simulink model "Spring_Test"  (R2025a)
settings: Solver=ode23t  StartTime=0.0  StopTime=15  RelTol=1e-3  EnableMultiTasking=on
InitFcn:
  | warning off Simulink:SL_MatchingFromNotFound
  | m=1;
  | b=1;
  | k=1;
libraries: fl_lib x15, nesl_utility x4, Custom_lib x1
Description:
  | Copyright 2015-2025 The MathWorks, Inc.
settings Model: Creator=tegel  LastModifiedBy=smiller
settings SolverCC: AlgebraicLoopSolver=TrustRegion
settings DataIOCC: LimitDataPoints=on  SaveFormat=Array  SignalLoggingSaveFormat=ModelDataLogs  ReturnWorkspaceOutputs=off
settings OptimizationCC: ReuseModelBlockBuffer=off  ExpressionDepthLimit=2147483647.0  InitFltsAndDblsToZero=on  LifeSpan=inf
settings DebuggingCC: SaveWithParameterizedLinksMsg=none  UnderspecifiedInitializationDetection=Classic  MergeDetectMultiDrivingBlocksExec=none  FcnCallInpInsideContextMsg=warning  UnconnectedInputMsg=warning  UnconnectedOutputMsg=warning  UnconnectedLineMsg=warning  AllowSymbolicDim=off  StateNameClashWarn=warning  PregeneratedLibrarySubsystemCodeDiagnostic=none  SFUnexpectedBacktrackingDiag=warning  SFNoUnconditionalDefaultTransitionDiag=warning  SFExecutionAtInitializationDiag=none  ArithmeticOperatorsInVariantConditions=warning
settings HardwareCC: ProdBitPerPointer=32.0  ProdBitPerSizeT=32.0  ProdBitPerPtrDiffT=32.0  ProdLargestAtomicFloat=None  ProdIntDivRoundTo=Undefined  ProdEndianess=Unspecified  ProdWordSize=32.0  ProdHWDeviceType=32-bit Generic
settings ModelReferenceCC: EnableRefExpFcnMdlSchedulingChecks=on  PropagateSignalLabelsOutOfModel=off
settings SFSimCC: SimUseLocalCustomCode=off  CustomCodeUndefinedFunction=UseInterfaceOnly
settings RTWCC: RTWUseLocalCustomCode=off  GPUComputeCapability=3.5  DLArmComputeVersion=19.05
settings CodeAppCC: StateflowObjectComments=on
settings GRTTargetCC: TargetFcnLib=ansi_tfl_tmw.mat  TargetLangStandard=C89/C90 (ANSI)  CombineOutputUpdateFcns=off  GRTInterface=on
settings ConfigComp: CovMetricSettings=dw  CovSaveCumulativeToWorkspaceVar=on  CovSaveSingleToWorkspaceVar=on  CovExternalEMLEnable=off  CovSFcnEnable=off
settings SimscapeCC: SimscapeNormalizeSystem=off  SimscapeNominalValues="[{\"value\":\"10\",\"unit\":\"V\"},{\"value\":\"1\",\"unit\":\"A\"},{\"value\":\"10\",\"unit\":\"N*m\"},{\"value\":\"10\",\"unit\":\"bar\"},{\"value\":\"100\",\"unit\":\"kJ/kg\"},{\"value\":\"1\",\"unit\":\"kW\"},{\"value\":\"300\",\"unit\":\"K\"},{\"value\":\"100\",\"unit\":\"cm^3/s\"},{\"value\":\"1\",\"unit\":\"kN\"},{\"value\":\"1\",\"unit\":\"g/cm^3\"},{\"value\":\"1\",\"unit\":\"l\"},{\"value\":\"1\",\"unit\":\"cm^2\"},{\"value\":\"60\",\"unit\":\"Hz\"}]"

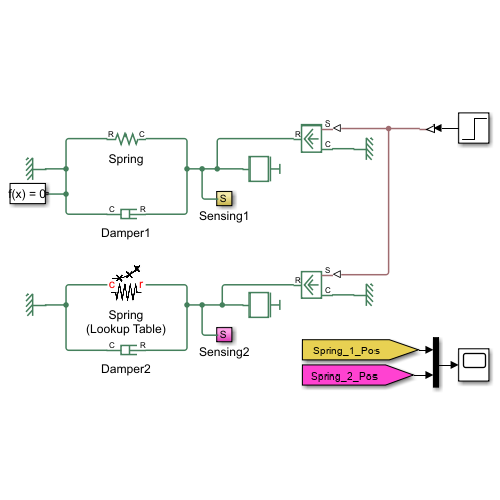
[thumbnail: Simulink's stored preview of the top-level diagram]
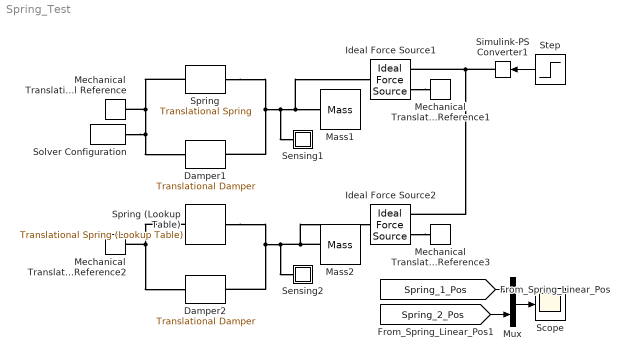
== system Spring_Test ==
  Damper1 : fl_lib/Mechanical/Translational Elements/Translational Damper  D=b N/(m/s)  v_specify=off  v_priority=High  v=0 m/s  v_nominal_specify=off  v_nominal_value=1  v_nominal_unit=m/s  f_specify=off  f_priority=High  f=0 N  f_nominal_specify=off  f_nominal_value=1  f_nominal_unit=N
  Damper2 : fl_lib/Mechanical/Translational Elements/Translational Damper  D=b N/(m/s)  v_specify=off  v_priority=High  v=0 m/s  v_nominal_specify=off  v_nominal_value=1  v_nominal_unit=m/s  f_specify=off  f_priority=High  f=0 N  f_nominal_specify=off  f_nominal_value=1  f_nominal_unit=N
  Ideal Force Source1 : fl_lib/Mechanical/Mechanical Sources/Ideal Force Source
  Ideal Force Source2 : fl_lib/Mechanical/Mechanical Sources/Ideal Force Source
  Mass1 : fl_lib/Mechanical/Translational Elements/Mass  mass=m kg  num_ports=foundation.enum.numPorts2.one  v_specify=on  v_priority=High  v=0 m/s  v_nominal_specify=off  v_nominal_value=1  v_nominal_unit=m/s  f_specify=off  f_priority=High  f=0 N  f_nominal_specify=off  f_nominal_value=1  f_nominal_unit=N
  Mass2 : fl_lib/Mechanical/Translational Elements/Mass  mass=m kg  num_ports=foundation.enum.numPorts2.one  v_specify=on  v_priority=High  v=0 m/s  v_nominal_specify=off  v_nominal_value=1  v_nominal_unit=m/s  f_specify=off  f_priority=High  f=0 N  f_nominal_specify=off  f_nominal_value=1  f_nominal_unit=N
  Mechanical Translational Reference{,1..3} (4 alike) : fl_lib/Mechanical/Translational Elements/Mechanical Translational Reference
  Mux : Mux  Inputs=2
  Scope : Scope
      settings: TimeSpan=15  ActiveDisplayYMinimum=-0.10033  ActiveDisplayYMaximum=0.90294
  Sensing1 : Subsystem
  Sensing2 : Subsystem
  Simulink-PS Converter1 : nesl_utility/Simulink-PS Converter  PhysicalDomain=network_engine_domain  SubClassName=ps_input  LeftPortType=input  RightPortType=output  PseudoPeriodic=off  Frequencies=[]  NoiseDistribution=none  NoiseParameters=[]  Unit=1  AffineConversion=off  FilteringAndDerivatives=zero  SimscapeFilterOrder=1  InputFilterTimeConstant=0.005  UdotUserProvided=0
  Solver Configuration : nesl_utility/Solver Configuration  PhysicalDomain=network_engine_domain  SubClassName=solver  LeftPortType=input  RightPortType=generic  Tones=[]  Harmonics=[]  SimulateNoise=off  Profile=off  UseLocalSampling=off  EnableSwitchedLinearOptims=on  FrequencyDomain=off  UseCCode=off  RelTol=0.001  AbsTol=1e-06  MinStep=1e-09  ToWorkspace=off  RevertToSquareIcSolve=off  NumHomotopyIterations=100  PhasorMode=off  PhasorModeNumHarmonics=1  ConsistencySolver=NEWTON_FTOL  IndexReductionMethod=DerivativeReplacement  DoDC=off  ResidualTolerance=1e-9  ConsistencyTolSource=GLOBAL  ConsistencyAbsTol=0.001  ConsistencyRelTol=0.001  ConsistencyTolFactor=0.001  UseLocalSolver=off  LocalSolverChoice=NE_BACKWARD_EULER_ADVANCER  ResolveIndetEquations=on  FunctionEvalNumThread=1  LocalSolverSampleTime=.001  DoFixedCost=off  MaxNonlinIter=12  MaxModeIter=2  ComputeImpulses=off  ImpulseIterations=2  LinearAlgebra=Sparse  LinearAlgebraNumThread=0  EquationFormulation=NE_TIME_EF  DelaysMemoryBudget=1024  AutomaticFiltering=on  FilteringTimeConstant=0.001  PartitionStorageMethod=AS_NEEDED  PartitionMemoryBudget=1024  PartitionMethod=FAST  MultibodyUseLocalSolver=off  MultibodyLocalSolverChoice=ODE1  MultibodyLocalSolverSampleTime=0.001
  Spring : fl_lib/Mechanical/Translational Elements/Translational Spring  spr_rate=10 N/m  v_specify=off  v_priority=High  v=0 m/s  v_nominal_specify=off  v_nominal_value=1  v_nominal_unit=m/s  f_specify=off  f_priority=High  f=0 N  f_nominal_specify=off  f_nominal_value=1  f_nominal_unit=N  x_specify=on  x_priority=High  x=0 m  x_nominal_specify=off  x_nominal_value=1  x_nominal_unit=m
  Spring (Lookup Table) : Custom_lib/Mechanical/Translational Spring (Lookup Table)  xd=[ -0.5 -0.4 0 0.4 0.5] mm  kd=[50 10 10 10 50] N/m  f_specify=off  f_priority=High  f=0 N  f_nominal_specify=off  f_nominal_value=1  f_nominal_unit=N  x_specify=off  x_priority=High  x=0 m  x_nominal_specify=off  x_nominal_value=1  x_nominal_unit=m  v_specify=off  v_priority=High  v=0 m/s  v_nominal_specify=off  v_nominal_value=1  v_nominal_unit=m/s  k_specify=off  k_priority=High  k=0 N/m  k_nominal_specify=off  k_nominal_value=1  k_nominal_unit=N/m
      settings: InternalSimscapePortConfiguration="{\"Bottom\":[],\"Left\":[{\"id\":\"c\",\"label\":\"c\",\"type\":\"foundation.mechanical.translational.translational\"}],\"Right\":[{\"id\":\"r\",\"label\":\"r\",\"type\":\"foundation.mechanical.translational.translational\"}],\"Top\":[]}"
  Step : Step  After=5e-3  SampleTime=0
  wires:
  Mux/1 -> Scope/1
  [Spring_1_Pos] -> Mux/1
  [Spring_2_Pos] -> Mux/2
  Step/1 -> Simulink-PS Converter1/1
  connections:
  Simulink-PS Converter1/RConn1 -- Ideal Force Source1/RConn1 -- Ideal Force Source2/RConn1
  Ideal Force Source1/RConn2 -- Mechanical Translational Reference1/LConn1
  Spring/LConn1 -- Mechanical Translational Reference/LConn1 -- Damper1/RConn1 -- Solver Configuration/RConn1
  Spring/RConn1 -- Damper1/LConn1 -- Sensing1/LConn1 -- Mass1/LConn1 -- Ideal Force Source1/LConn1
  Mechanical Translational Reference2/LConn1 -- Spring (Lookup Table)/LConn1 -- Damper2/RConn1
  Damper2/LConn1 -- Spring (Lookup Table)/RConn1 -- Sensing2/LConn1 -- Mass2/LConn1 -- Ideal Force Source2/LConn1
  Ideal Force Source2/RConn2 -- Mechanical Translational Reference3/LConn1

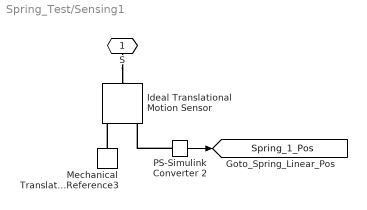
== system Spring_Test/Sensing1 ==
  Ideal Translational Motion Sensor : fl_lib/Mechanical/Mechanical Sensors/Ideal Translational Motion Sensor  reference=foundation.enum.MeasurementReference.difference  acceleration_port=false  velocity_port=true  position_port=true  offset=0 m
  Mechanical Translational Reference3 : fl_lib/Mechanical/Translational Elements/Mechanical Translational Reference
  PS-Simulink Converter 2 : nesl_utility/PS-Simulink Converter  PhysicalDomain=network_engine_domain  SubClassName=ps_output  LeftPortType=input  RightPortType=output  PseudoPeriodic=off  Frequencies=[]  VectorFormat=1-D array  Unit=mm  AffineConversion=off
  S : PMIOPort  Side=Left
  tag scope: Spring_1_Pos=global
  wires:
  PS-Simulink Converter 2/1 -> [Spring_1_Pos]
  connections:
  S/RConn1 -- Ideal Translational Motion Sensor/LConn1
  Mechanical Translational Reference3/LConn1 -- Ideal Translational Motion Sensor/RConn1
  PS-Simulink Converter 2/LConn1 -- Ideal Translational Motion Sensor/RConn3

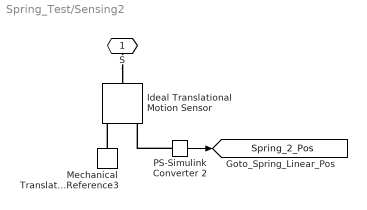
== system Spring_Test/Sensing2 ==
  Ideal Translational Motion Sensor : fl_lib/Mechanical/Mechanical Sensors/Ideal Translational Motion Sensor  reference=foundation.enum.MeasurementReference.difference  acceleration_port=false  velocity_port=true  position_port=true  offset=0 m
  Mechanical Translational Reference3 : fl_lib/Mechanical/Translational Elements/Mechanical Translational Reference
  PS-Simulink Converter 2 : nesl_utility/PS-Simulink Converter  PhysicalDomain=network_engine_domain  SubClassName=ps_output  LeftPortType=input  RightPortType=output  PseudoPeriodic=off  Frequencies=[]  VectorFormat=1-D array  Unit=mm  AffineConversion=off
  S : PMIOPort  Side=Left
  tag scope: Spring_2_Pos=global
  wires:
  PS-Simulink Converter 2/1 -> [Spring_2_Pos]
  connections:
  PS-Simulink Converter 2/LConn1 -- Ideal Translational Motion Sensor/RConn3
  Mechanical Translational Reference3/LConn1 -- Ideal Translational Motion Sensor/RConn1
  S/RConn1 -- Ideal Translational Motion Sensor/LConn1
